simulink model "tb_lvservomtr_open_loop"  (R2025b)
settings: Solver=VariableStepAuto  StartTime=0.0  StopTime=0.08  RelTol=1e-3
settings Model: Creator=semih  LastModifiedBy=semih

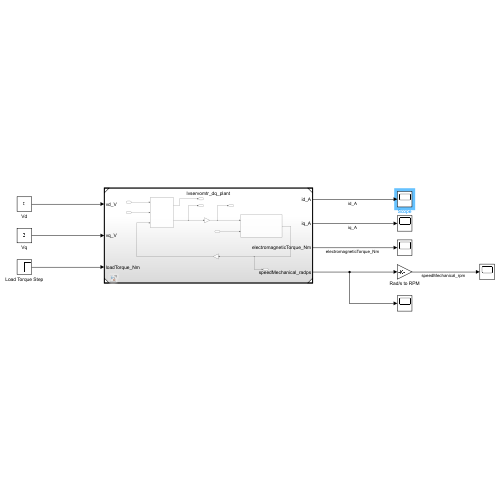
[thumbnail: Simulink's stored preview of the top-level diagram]
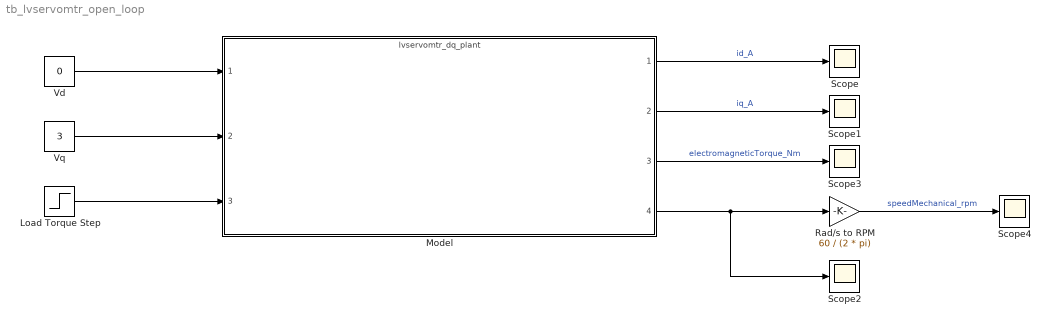
== system tb_lvservomtr_open_loop ==
  Load Torque Step : Step  Time=0.030  After=0.05  SampleTime=0
  Model : ModelReference  ModelNameDialog=lvservomtr_dq_plant  SimulationMode=Normal  ModelReferenceVersion=1.7
  Rad/s to RPM : Gain  Gain=60 / (2 * pi)
  Scope{,1..4} (5 alike) : Scope
      Scope settings: ActiveDisplayYMinimum=-0.42366511792142403  ActiveDisplayYMaximum=1.8876545573518515
      Scope1 settings: ActiveDisplayYMinimum=-0.782694880235963  ActiveDisplayYMaximum=7.0442539221236693
      Scope2 settings: ActiveDisplayYMinimum=-14.648422716149396  ActiveDisplayYMaximum=131.83580444534459  DataLoggingVariableName=ScopeData2
      Scope3 settings: ActiveDisplayYMinimum=-0.077109095292808  ActiveDisplayYMaximum=0.69398185763527209  DataLoggingVariableName=ScopeData3
      Scope4 settings: ActiveDisplayYMinimum=-139.88213302648705  ActiveDisplayYMaximum=1258.9391972383837  DataLoggingVariableName=ScopeData4
  Vd : Constant  Value=0
  Vq : Constant  Value=3
  wires:
  Load Torque Step/1 -> Model/3
  Rad/s to RPM/1 -> Scope4/1  "speedMechanical_rpm"
  Model/4 -> Scope2/1, Rad/s to RPM/1
  Vq/1 -> Model/2
  Vd/1 -> Model/1
  Model/3 -> Scope3/1  "electromagneticTorque_Nm"
  Model/1 -> Scope/1  "id_A"
  Model/2 -> Scope1/1  "iq_A"
